simulink model "test_LQI_psi"  (R2025b)
settings: Solver=VariableStepAuto  StartTime=0.0  StopTime=30  RelTol=1e-3
values from neighbouring files (symbols this model uses):
  Kd = 0.8 * K_aug(2)    [gains_LQI.m]
  Kd_psi = K_aug_psi(2)    [gains_LQI.m]
  Ki = 0.8 * K_aug(3)    [gains_LQI.m]
  Ki_psi = K_aug_psi(3)    [gains_LQI.m]
  Kp = 0.8 * K_aug(1)    [gains_LQI.m]
  Kp_psi = K_aug_psi(1)    [gains_LQI.m]
  tau = 1.2    [gains_LQI.m]
undefined symbols (not defined in the file or in its folder): DiscIntNeverNeededParam
libraries: simulink x2
settings Model: Creator=anoua  LastModifiedBy=anoua

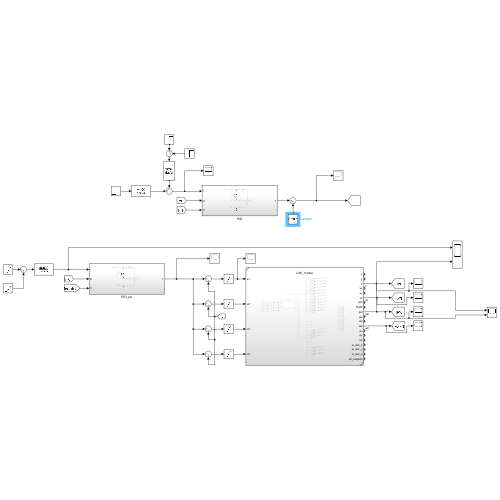
[thumbnail: Simulink's stored preview of the top-level diagram]
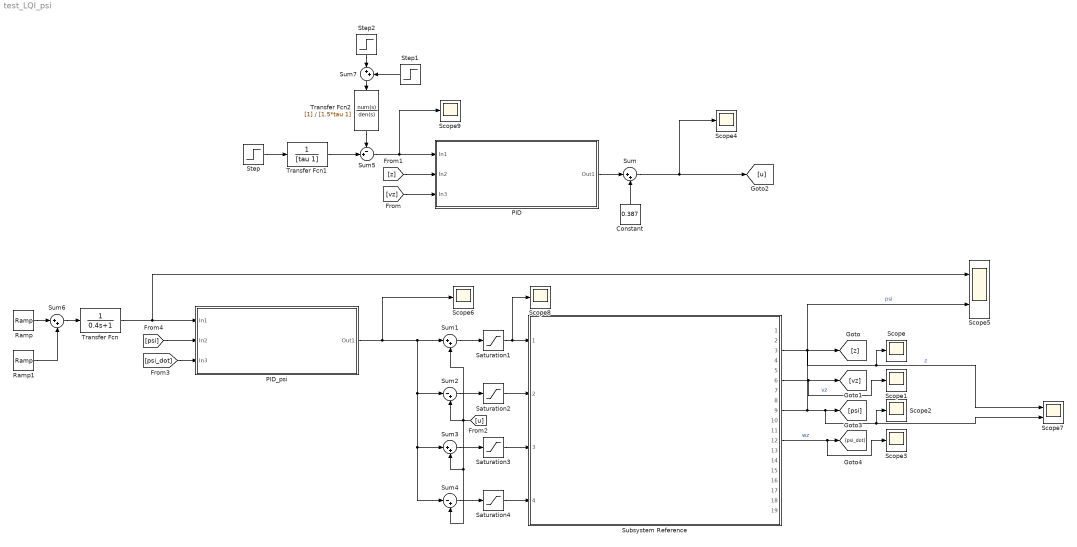
== system test_LQI_psi ==
  Constant : Constant  Value=0.387
  PID : Subsystem
  PID_psi : Subsystem
  Ramp : simulink/Sources/Ramp  slope=18  start=5  InitialOutput=0
  Ramp1 : simulink/Sources/Ramp  slope=-18  start=15  InitialOutput=0
  Saturation{1..4} (4 alike) : Saturate  UpperLimit=1  LowerLimit=-1
  Scope{,1..4,6,8..9} (8 alike) : Scope
      Scope settings: ActiveDisplayYMinimum=-0.52568434481368709  ActiveDisplayYMaximum=0.7726511161711308
      Scope1 settings: ActiveDisplayYMinimum=-1.3340291702690279  ActiveDisplayYMaximum=1.1408884147091976
      Scope2 settings: ActiveDisplayYMinimum=-22.80887139572668  ActiveDisplayYMaximum=205.26585926668622  DataLoggingVariableName=ScopeData2
      Scope3 settings: ActiveDisplayYMinimum=-2.4296027110352618  ActiveDisplayYMaximum=20.369635182782769  DataLoggingVariableName=ScopeData5
      Scope4 settings: ActiveDisplayYMinimum=0.37906499640827757  ActiveDisplayYMaximum=0.40083244418879344  DataLoggingVariableName=ScopeData4
      Scope6 settings: ActiveDisplayYMinimum=-0.22428640967526348  ActiveDisplayYMaximum=0.23402768902565715  DataLoggingVariableName=ScopeData7
      Scope8 settings: ActiveDisplayYMinimum=-0.10711700708251803  ActiveDisplayYMaximum=1.1088445409943304  DataLoggingVariableName=ScopeData9
      Scope9 settings: ActiveDisplayYMinimum=-0.643410170889133  ActiveDisplayYMaximum=0.715551218048372  DataLoggingVariableName=ScopeData10
  Scope5 : Scope  NumInputPorts=2
      settings: ActiveDisplayYMinimum=-22.80887139572668  ActiveDisplayYMaximum=205.26585926668622  DataLoggingVariableName=ScopeData6
  Scope7 : Scope  NumInputPorts=2
      settings: ActiveDisplayYMinimum=-1  ActiveDisplayYMaximum=1  DataLoggingVariableName=ScopeData8
  Step : Step  Time=0  After=0.5  SampleTime=0
  Step1 : Step  Time=16  After=0.70  SampleTime=0
  Step2 : Step  Time=22  After=0.05  SampleTime=0
  Subsystem Reference : Subsystem  ReferencedSubsystem=UAV_model
  Sum{,1,3,6..7} (5 alike) : Sum  Inputs=|++
  Sum2 : Sum  Inputs=|-+
  Sum4 : Sum  Inputs=|-+
  Sum5 : Sum  Inputs=-+|
  Transfer Fcn : TransferFcn  Denominator=[0.4 1]
  Transfer Fcn1 : TransferFcn  Denominator=[tau 1]
  Transfer Fcn2 : TransferFcn  Denominator=[1.5*tau 1]
  wires:
  Subsystem Reference/3 -> Scope7/1, Scope/1, [z]  "z"
  Subsystem Reference/6 -> Scope1/1, [vz]  "vz"
  PID/1(Out1) -> Sum/1
  [vz] -> PID/3(In3)
  [z] -> PID/2(In2)
  Sum1/1 -> Saturation1/1
  Sum2/1 -> Saturation2/1
  Sum3/1 -> Saturation3/1
  Sum4/1 -> Saturation4/1
  [u] -> Sum4/2, Sum3/2, Sum1/2, Sum2/2
  Sum/1 -> [u], Scope4/1
  PID_psi/1(Out1) -> Sum1/1, Sum3/1, Sum4/1, Sum2/1, Scope6/1
  [psi_dot] -> PID_psi/3(In3)
  [psi] -> PID_psi/2(In2)
  Subsystem Reference/9 -> Scope7/2, Scope2/1, [psi], Scope5/2  "psi"
  Subsystem Reference/12 -> [psi_dot], Scope3/1  "wz"
  Ramp/1 -> Sum6/1
  Sum6/1 -> Transfer Fcn/1
  Ramp1/1 -> Sum6/2
  Transfer Fcn/1 -> Scope5/1, PID_psi/1(In1)
  Saturation1/1 -> Scope8/1, Subsystem Reference/1
  Saturation2/1 -> Subsystem Reference/2
  Saturation3/1 -> Subsystem Reference/3
  Saturation4/1 -> Subsystem Reference/4
  Step/1 -> Transfer Fcn1/1
  Transfer Fcn1/1 -> Sum5/2
  Transfer Fcn2/1 -> Sum5/1
  Sum7/1 -> Transfer Fcn2/1
  Step1/1 -> Sum7/2
  Step2/1 -> Sum7/1
  Sum5/1 -> Scope9/1, PID/1(In1)
  Constant/1 -> Sum/2

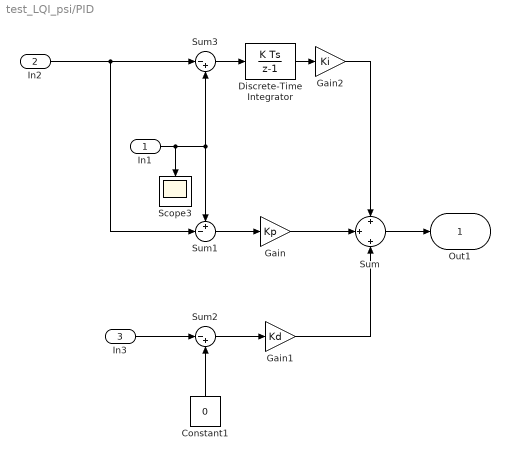
== system test_LQI_psi/PID ==
  In1 : Inport
  In2 : Inport  Port=2
  In3 : Inport  Port=3
  Constant1 : Constant  Value=0
  Discrete-Time Integrator : DiscreteIntegrator  SampleTime=-1  LimitOutput=on  UpperSaturationLimit=1/Ki  LowerSaturationLimit=-1/Ki  ICPrevOutput=DiscIntNeverNeededParam  ICPrevScaledInput=DiscIntNeverNeededParam
  Gain : Gain  Gain=Kp
  Gain1 : Gain  Gain=Kd
  Gain2 : Gain  Gain=Ki
  Scope3 : Scope
      settings: ActiveDisplayYMinimum=-0.53484809981403014  ActiveDisplayYMaximum=1.6271171549271228  DataLoggingVariableName=ScopeData3
  Sum : Sum  Inputs=+|+|+
  Sum1 : Sum  Inputs=+-|
  Sum2 : Sum  Inputs=|-+
  Sum3 : Sum  Inputs=|-+
  Out1 : Outport
  wires:
  Gain2/1 -> Sum/1
  Gain/1 -> Sum/2
  Sum2/1 -> Gain1/1
  Gain1/1 -> Sum/3
  In1/1 -> Sum3/2, Sum1/1, Scope3/1
  Sum1/1 -> Gain/1
  Discrete-Time Integrator/1 -> Gain2/1
  Constant1/1 -> Sum2/2
  Sum3/1 -> Discrete-Time Integrator/1
  Sum/1 -> Out1/1
  In2/1 -> Sum1/2, Sum3/1
  In3/1 -> Sum2/1

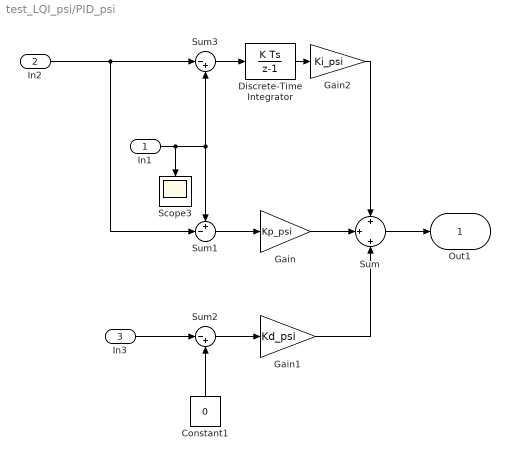
== system test_LQI_psi/PID_psi ==
  In1 : Inport
  In2 : Inport  Port=2
  In3 : Inport  Port=3
  Constant1 : Constant  Value=0
  Discrete-Time Integrator : DiscreteIntegrator  SampleTime=-1  LimitOutput=on  UpperSaturationLimit=1/Ki_psi  LowerSaturationLimit=-1/Ki_psi  ICPrevOutput=DiscIntNeverNeededParam  ICPrevScaledInput=DiscIntNeverNeededParam
  Gain : Gain  Gain=Kp_psi
  Gain1 : Gain  Gain=Kd_psi
  Gain2 : Gain  Gain=Ki_psi
  Scope3 : Scope
      settings: ActiveDisplayYMinimum=-0.53484809981403014  ActiveDisplayYMaximum=1.6271171549271228  DataLoggingVariableName=ScopeData3
  Sum : Sum  Inputs=+|+|+
  Sum1 : Sum  Inputs=+-|
  Sum2 : Sum  Inputs=|-+
  Sum3 : Sum  Inputs=|-+
  Out1 : Outport
  wires:
  Gain2/1 -> Sum/1
  Gain/1 -> Sum/2
  Sum2/1 -> Gain1/1
  Gain1/1 -> Sum/3
  In1/1 -> Sum3/2, Sum1/1, Scope3/1
  Sum1/1 -> Gain/1
  Discrete-Time Integrator/1 -> Gain2/1
  Constant1/1 -> Sum2/2
  Sum3/1 -> Discrete-Time Integrator/1
  Sum/1 -> Out1/1
  In2/1 -> Sum1/2, Sum3/1
  In3/1 -> Sum2/1
